simulink model "RealseCheckPWMController"  (R2026a)
settings: Solver=ode4  StopTime=inf  FixedStep=1/500  EnableMultiTasking=on
undefined symbols (not defined in the file): HIL, qc_get_step_size
libraries: quarc_library x12
settings Model: SimulationMode=external  ExtModeTrigDuration=10000  Creator=fvranes  LastModifiedBy=meow1
settings SolverCC: PositivePriorityOrder=on
settings RTWCC: SystemTargetFile=quarc_win64.tlc  TemplateMakefile=quarc_default_tmf  Toolchain=QUARC win64 | nmake (64-bit Windows)  BuildConfiguration=Faster Runs  Description=QUARC Win64 Target Using Toolchain
settings STFCustomTargetCC: SystemTargetFile=quarc_win64.tlc  MultiwordLength=2048.0  ConcurrentExecutionCompliant=on  UseToolchainInfoCompliant=on
settings GRTTargetCC: ExtMode=on  ExtModeMexFile=quarc_comm  ParMdlRefBuildCompliant=off  CompOptLevelCompliant=off  CombineOutputUpdateFcns=off  MatFileLogging=off  CPPClassGenCompliant=off  GRTInterface=on
settings ConfigComp: CovMetricSettings=dswe

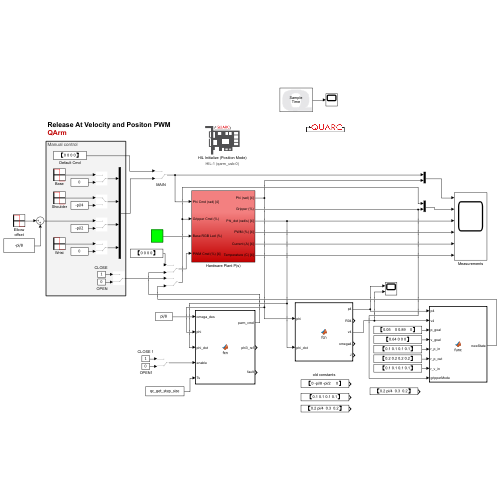
[thumbnail: Simulink's stored preview of the top-level diagram]
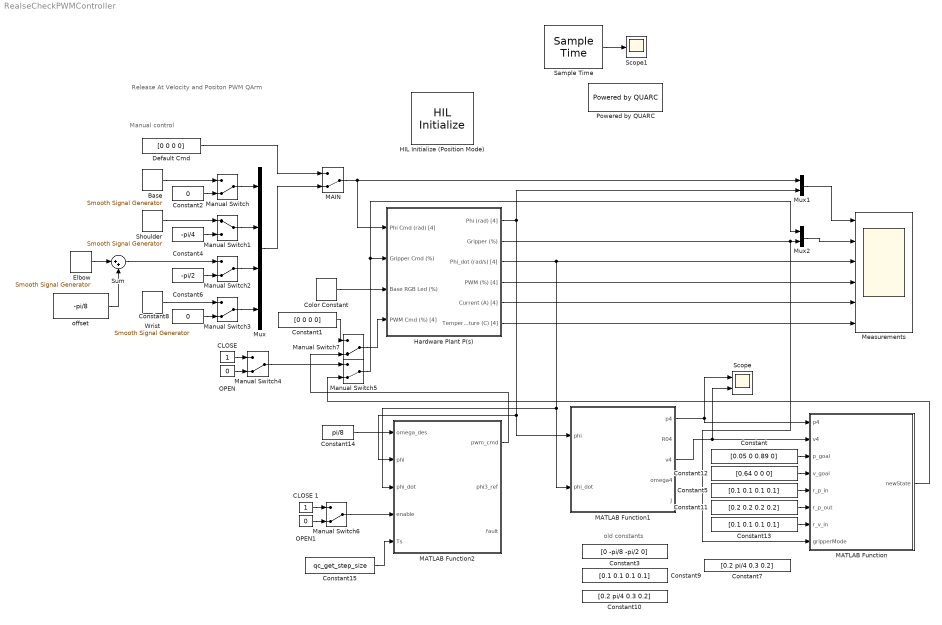
== system RealseCheckPWMController ==
  note: old constants
  note: Manual control
  note: Release At Velocity and Positon PWM
      | QArm
  " OPEN" : Constant  Value=0
  " OPEN1" : Constant  Value=0
  Base : quarc_library/Sources/Signals/Smooth Signal Generator  signal_type=Square  source=Internal (dialog parameters)  amplitude=pi/8  frequency=0.125  initial_phase=0  sample_time=qc_get_step_size  output_cos=off
      settings: SourceProductName=QUARC Targets
  "CLOSE " : Constant
  CLOSE 1 : Constant
  Color Constant : quarc_library/Sources/Signals/Color Constant  color=[0 1 0]
      settings: SourceProductName=QUARC Targets
  Constant : Constant  Value=[0.05 0 0.89 0]
  Constant1 : Constant  Value=[0 0 0 0]
  Constant10 : Constant  Value=[0.2 pi/4 0.3 0.2]
  Constant11 : Constant  Value=[0.2 0.2 0.2 0.2]
  Constant12 : Constant  Value=[0.64 0 0 0]
  Constant13 : Constant  Value=[0.1 0.1 0.1 0.1]
  Constant14 : Constant  Value=pi/8
  Constant15 : Constant  Value=qc_get_step_size
  Constant2 : Constant  Value=0
  Constant3 : Constant  Value=[0 -pi/8 -pi/2 0]
  Constant4 : Constant  Value=-pi/4
  Constant5 : Constant  Value=[0.1 0.1 0.1 0.1]
  Constant6 : Constant  Value=-pi/2
  Constant7 : Constant  Value=[0.2 pi/4 0.3 0.2]
  Constant8 : Constant  Value=0
  Constant9 : Constant  Value=[0.1 0.1 0.1 0.1]
  Default Cmd : Constant  Value=[0 0 0 0]
  Elbow : quarc_library/Sources/Signals/Smooth Signal Generator  signal_type=Square  source=Internal (dialog parameters)  amplitude=pi/4  frequency=0.25  initial_phase=pi  sample_time=qc_get_step_size  output_cos=off
      settings: SourceProductName=QUARC Targets
  HIL Initialize (Position Mode) : quarc_library/Data Acquisition/Generic/Configuration/HIL Initialize  object_name=HIL-1  board_type=qarm_usb  board_number=0  board_options=j0_mode=0;j1_mode=0;j2_mode=1;j3_mode=0;gripper_mode=0;j0_profile_config=0;j0_profile_velocity=1.6;j0_profile_acceleration=1.0472;j1_profile_config=0;j1_profile_velocity=1.6;j1_profile_acceleration=1.0472;j2_profile_config=0;j2_profile_velocity=1.6;j2_profile_acceleration=1.0472;j3_profile_config=0;j3_profile_velocity=1.6;j3_profile_acceleration=1.0472;  exclusive=off  active=on  hardware_clocks=[0]  clock_modes=[]  initial_clock_frequencies=[]  set_clock_params_at_start=off  set_clock_params_at_switch_in=off  set_clock_frequencies_at_start=off  set_clock_frequencies_at_switch_in=off  analog_input_channels=[5:9]  analog_input_configurations=[]  analog_input_maximums=[]  analog_input_minimums=[]  set_analog_input_params_at_start=off  set_analog_input_params_at_switch_in=off  analog_output_channels=[]  analog_output_maximums=inf  analog_output_minimums=-inf  initial_analog_outputs=[0]  final_analog_outputs=[0]  watchdog_analog_outputs=[]  set_analog_output_params_at_start=off  set_analog_output_params_at_switch_in=off  set_analog_outputs_at_start=off  set_analog_outputs_at_switch_in=off  set_analog_outputs_at_terminate=off  set_analog_outputs_at_switch_out=off  set_analog_outputs_on_watchdog=off  digital_input_channels=[]  digital_output_channels=[]  digital_output_configuration=[]  initial_digital_outputs=[0]  final_digital_outputs=[0]  watchdog_digital_outputs=[0]  set_digital_output_params_at_start=off  set_digital_output_params_at_switch_in=off  set_digital_outputs_at_start=off  set_digital_outputs_at_switch_in=off  set_digital_outputs_at_terminate=off  set_digital_outputs_at_switch_out=off  set_digital_outputs_on_watchdog=off  encoder_channels=[]  quadrature=[]  encoder_filter_frequency=[]  initial_encoder_counts=[]  set_encoder_params_at_start=off  set_encoder_params_at_switch_in=off  set_encoder_counts_at_start=off  set_encoder_counts_at_switch_in=off  pwm_channels=[]  pwm_modes=[]  pwm_frequency=[]  pwm_configuration=[]  pwm_alignment=[]  pwm_polarity=[]  pwm_leading_deadband=[]  pwm_trailing_deadband=[]  initial_pwm_outputs=[]  final_pwm_outputs=[]  watchdog_pwm_outputs=[]  set_pwm_params_at_start=off  set_pwm_params_at_switch_in=off  set_pwm_outputs_at_start=off  set_pwm_outputs_at_switch_in=off  set_pwm_outputs_at_terminate=off  set_pwm_outputs_at_switch_out=off  set_pwm_outputs_on_watchdog=off  other_output_channels=[11005:11008 1000:1004 11000:11003]  initial_other_outputs=[zeros(1,9), ones(1,3)]  final_other_outputs=[1 0 0 0]  watchdog_other_outputs=zeros(1,12)  set_other_outputs_at_start=off  set_other_outputs_at_switch_in=off  set_other_outputs_at_terminate=on  set_other_outputs_at_switch_out=off  set_other_outputs_on_watchdog=off
  Hardware Plant P(s) : Subsystem
  MAIN : ManualSwitch  CurrentSetting=0
  MATLAB Function : MATLAB Function  TreatAsAtomicUnit=on
  MATLAB Function1 : MATLAB Function  TreatAsAtomicUnit=on
  MATLAB Function2 : MATLAB Function  TreatAsAtomicUnit=on
  Manual Switch{,2..7} (7 alike) : ManualSwitch  CurrentSetting=0
  Manual Switch1 : ManualSwitch
  Measurements : Scope  NumInputPorts=6
      settings: TimeSpan=20  Title=Phi (angular position)  ActiveDisplayYMinimum=-3.0435003762492152  ActiveDisplayYMaximum=0.767085796973318  YLabel=degrees
  Mux : Mux
  Mux1 : Mux  Inputs=2
  Mux2 : Mux  Inputs=2
  Powered by QUARC : quarc_library/Logos/Powered by QUARC
  Sample Time : quarc_library/Sources/Time/Sample Time  Priority=-99  sample_time=qc_get_step_size
  Scope : Scope  NumInputPorts=2
      settings: DataLoggingVariableName=ScopeData2
  Scope1 : Scope
      settings: ActiveDisplayYMinimum=0.00125  ActiveDisplayYMaximum=0.00274
  Shoulder : quarc_library/Sources/Signals/Smooth Signal Generator  signal_type=Square  source=Internal (dialog parameters)  amplitude=pi/3  frequency=0.25  initial_phase=0  sample_time=qc_get_step_size  output_cos=off
      settings: SourceProductName=QUARC Targets
  Sum : Sum  Inputs=|++
  Wrist : quarc_library/Sources/Signals/Smooth Signal Generator  signal_type=Square  source=Internal (dialog parameters)  amplitude=pi/8  frequency=0.125  initial_phase=0  sample_time=qc_get_step_size  output_cos=off
      settings: SourceProductName=QUARC Targets
  offset : Constant  Value=-pi/8
  wires:
  Color Constant/1 -> Hardware Plant P(s)/3(Base RGB Led (%))
  Constant2/1 -> Manual Switch/2
  Constant4/1 -> Manual Switch1/2
  Constant6/1 -> Manual Switch2/2
  Constant8/1 -> Manual Switch3/2
  Wrist/1 -> Manual Switch3/1
  Manual Switch2/1 -> Mux/3
  Manual Switch3/1 -> Mux/4
  Manual Switch1/1 -> Mux/2
  Manual Switch/1 -> Mux/1
  Mux/1 -> MAIN/2
  Default Cmd/1 -> MAIN/1
  MAIN/1 -> Mux1/1, Hardware Plant P(s)/1(Phi Cmd (rad) [4])
  "CLOSE "/1 -> Manual Switch4/1
  Base/1 -> Manual Switch/1
  Shoulder/1 -> Manual Switch1/1
  Elbow/1 -> Sum/1
  Sample Time/1 -> Scope1/1
  " OPEN"/1 -> Manual Switch4/2
  Hardware Plant P(s)/2(Gripper (%)) -> Mux2/2, MATLAB Function/8(gripperMode)
  Constant/1 -> MATLAB Function/3(p_goal)
  Constant5/1 -> MATLAB Function/5(r_p_in)
  Hardware Plant P(s)/1(Phi (rad) [4]) -> MATLAB Function2/2(phi), MATLAB Function1/1(phi), Mux1/2
  Hardware Plant P(s)/3(Phi_dot (rad/s) [4]) -> MATLAB Function1/2(phi_dot), MATLAB Function2/3(phi_dot), Measurements/3
  Mux2/1 -> Measurements/2
  Mux1/1 -> Measurements/1
  Hardware Plant P(s)/4(PWM (%) [4]) -> Measurements/4
  Hardware Plant P(s)/5(Current (A) [4]) -> Measurements/5
  Hardware Plant P(s)/6(Temperature (C) [4]) -> Measurements/6
  Manual Switch4/1 -> Manual Switch5/1
  MATLAB Function/1(newState) -> Manual Switch5/2
  Manual Switch5/1 -> Mux2/1, Hardware Plant P(s)/2(Gripper Cmd (%))
  offset/1 -> Sum/2
  Sum/1 -> Manual Switch2/1
  MATLAB Function1/1(p4) -> Scope/1, MATLAB Function/1(p4)
  MATLAB Function1/3(v4) -> Scope/2, MATLAB Function/2(v4)
  Constant11/1 -> MATLAB Function/6(r_p_out)
  Constant12/1 -> MATLAB Function/4(v_goal)
  Constant13/1 -> MATLAB Function/7(r_v_in)
  Constant14/1 -> MATLAB Function2/1(omega_des)
  CLOSE 1/1 -> Manual Switch6/1
  " OPEN1"/1 -> Manual Switch6/2
  Manual Switch6/1 -> MATLAB Function2/4(enable)
  Constant1/1 -> Manual Switch7/1
  MATLAB Function2/1(pwm_cmd) -> Manual Switch7/2
  Manual Switch7/1 -> Hardware Plant P(s)/4(PWM Cmd (%) [4])
  Constant15/1 -> MATLAB Function2/5(Ts)

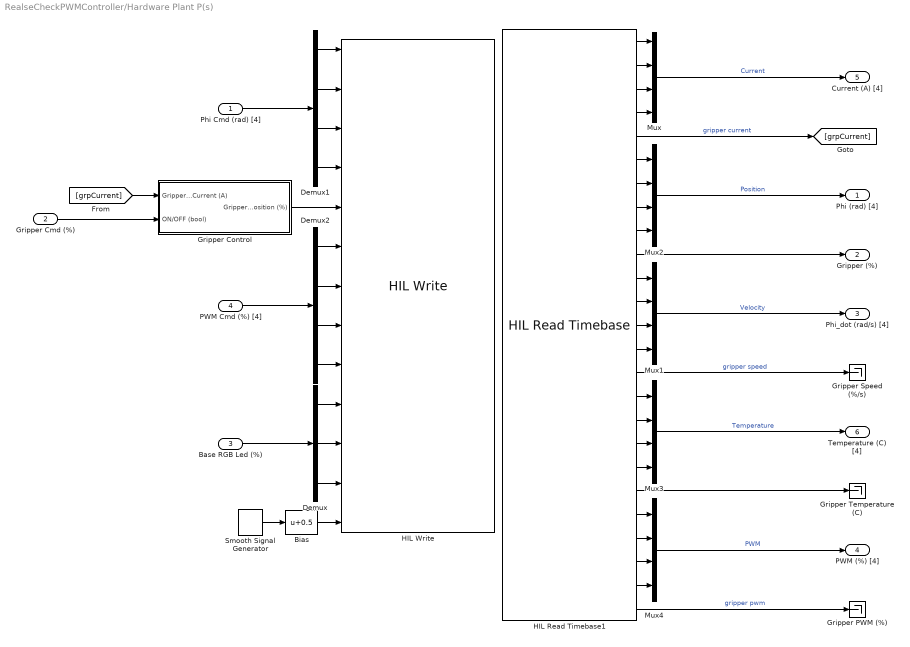
== system RealseCheckPWMController/Hardware Plant P(s) ==
  Phi Cmd (rad) [4] : Inport
  Gripper Cmd (%) : Inport  Port=2
  Base RGB Led (%) : Inport  Port=3
  PWM Cmd (%) [4] : Inport  Port=4
  Bias : Bias  Bias=0.5  SaturateOnIntegerOverflow=off
  Demux : Demux  Outputs=3
  Demux1 : Demux
  Demux2 : Demux
  Gripper Control : Subsystem
  Gripper PWM (%) : Terminator
  Gripper Speed (%/s) : Terminator
  Gripper Temperature (C) : Terminator
  HIL Read Timebase1 : quarc_library/Data Acquisition/Generic/Timebases/HIL Read Timebase  object_name=HIL-1  clock=0  analog_channels=[5:9]  encoder_channels=[]  digital_channels=[]  other_channels=[1000:1004 3000:3004 10000:10004 11000:11004]  active=on  vector_output=off  port_labels=channel numbers  data_type_mode=Inherit via back propagation  encoder_data_type=double  digital_data_type=boolean  overflow_mode=Error on overflow  samples_in_buffer=max(ceil(1/qc_get_step_size), 1)
  HIL Write : quarc_library/Data Acquisition/Generic/Immediate I//O/HIL Write  object_name=HIL-1  analog_channels=[]  pwm_channels=[]  digital_channels=[]  other_channels=[1000:1004 11000:11003 11005:11008]  sample_time=-1  active=on  vector_input=off  port_labels=channel numbers
  Mux{,1..4} (5 alike) : Mux
  Smooth Signal Generator : quarc_library/Sources/Signals/Smooth Signal Generator  signal_type=Sine  source=Internal (dialog parameters)  amplitude=0.5  frequency=0.5  initial_phase=0  sample_time=qc_get_step_size  output_cos=off
      settings: SourceProductName=QUARC Targets
  Phi (rad) [4] : Outport  VectorParamsAs1DForOutWhenUnconnected=off
  Gripper (%) : Outport  Port=2  VectorParamsAs1DForOutWhenUnconnected=off
  Phi_dot (rad/s) [4] : Outport  Port=3  VectorParamsAs1DForOutWhenUnconnected=off
  PWM (%) [4] : Outport  Port=4  VectorParamsAs1DForOutWhenUnconnected=off
  Current (A) [4] : Outport  Port=5  VectorParamsAs1DForOutWhenUnconnected=off
  Temperature (C) [4] : Outport  Port=6  VectorParamsAs1DForOutWhenUnconnected=off
  wires:
  Gripper Cmd (%)/1 -> Gripper Control/2(ON/OFF (bool))
  HIL Read Timebase1/10 -> Gripper (%)/1
  Mux4/1 -> PWM (%) [4]/1  "PWM"
  HIL Read Timebase1/25 -> Gripper PWM (%)/1  "gripper pwm"
  HIL Read Timebase1/24 -> Mux4/4
  HIL Read Timebase1/23 -> Mux4/3
  HIL Read Timebase1/22 -> Mux4/2
  HIL Read Timebase1/21 -> Mux4/1
  Mux2/1 -> Phi (rad) [4]/1  "Position"
  Demux2/4 -> HIL Write/9
  Demux2/3 -> HIL Write/8
  Demux2/2 -> HIL Write/7
  Demux2/1 -> HIL Write/6
  PWM Cmd (%) [4]/1 -> Demux2/1
  Phi Cmd (rad) [4]/1 -> Demux1/1
  Demux1/4 -> HIL Write/4
  Demux1/3 -> HIL Write/3
  Demux1/2 -> HIL Write/2
  Demux1/1 -> HIL Write/1
  Base RGB Led (%)/1 -> Demux/1
  Mux3/1 -> Temperature (C) [4]/1  "Temperature"
  Mux1/1 -> Phi_dot (rad/s) [4]/1  "Velocity"
  Mux/1 -> Current (A) [4]/1  "Current"
  HIL Read Timebase1/20 -> Gripper Temperature (C)/1
  HIL Read Timebase1/1 -> Mux/1
  HIL Read Timebase1/2 -> Mux/2
  HIL Read Timebase1/13 -> Mux1/3
  Demux/2 -> HIL Write/11
  HIL Read Timebase1/19 -> Mux3/4
  Demux/1 -> HIL Write/10
  HIL Read Timebase1/11 -> Mux1/1
  HIL Read Timebase1/16 -> Mux3/1
  HIL Read Timebase1/17 -> Mux3/2
  HIL Read Timebase1/3 -> Mux/3
  Demux/3 -> HIL Write/12
  HIL Read Timebase1/15 -> Gripper Speed (%/s)/1  "gripper speed"
  HIL Read Timebase1/5 -> [grpCurrent]  "gripper current"
  HIL Read Timebase1/7 -> Mux2/2
  HIL Read Timebase1/4 -> Mux/4
  HIL Read Timebase1/12 -> Mux1/2
  HIL Read Timebase1/8 -> Mux2/3
  HIL Read Timebase1/18 -> Mux3/3
  HIL Read Timebase1/6 -> Mux2/1
  HIL Read Timebase1/9 -> Mux2/4
  HIL Read Timebase1/14 -> Mux1/4
  Smooth Signal Generator/1 -> Bias/1
  Bias/1 -> HIL Write/13
  Gripper Control/1(Gripper Position (%)) -> HIL Write/5
  [grpCurrent] -> Gripper Control/1(Gripper Current (A))

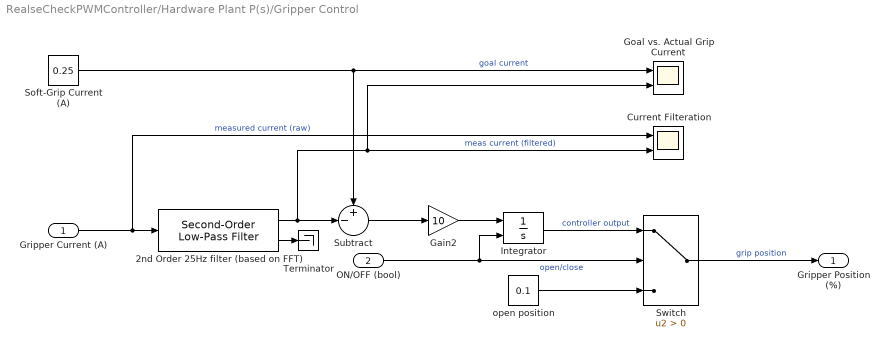
== system RealseCheckPWMController/Hardware Plant P(s)/Gripper Control ==
  Gripper Current (A) : Inport
  ON/OFF (bool) : Inport  Port=2
  2nd Order 25Hz filter (based on FFT) : quarc_library/Continuous/Second-Order Low-Pass Filter  params_source=Internal (dialog parameters)  input_width=25*2*pi  input_zeta=1  input_init=0
  Current Filteration : Scope  NumInputPorts=2
      settings: ActiveDisplayYMinimum=-0.01447  ActiveDisplayYMaximum=0.62651  DataLoggingVariableName=ScopeData5
  Gain2 : Gain  Gain=10
  Goal vs. Actual Grip Current : Scope  NumInputPorts=2
      settings: ActiveDisplayYMinimum=0.00229  ActiveDisplayYMaximum=0.27702  DataLoggingVariableName=ScopeData4
  Integrator : Integrator  ExternalReset=either  InitialCondition=0.1  LimitOutput=on  UpperSaturationLimit=0.9  LowerSaturationLimit=0.1
  Soft-Grip Current (A) : Constant  Value=0.25
  Subtract : Sum  Inputs=+-|
  Switch : Switch  Criteria=u2 > Threshold  SaturateOnIntegerOverflow=off  InputSameDT=off
  Terminator : Terminator
  open position : Constant  Value=0.1
  Gripper Position (%) : Outport  VectorParamsAs1DForOutWhenUnconnected=off
  wires:
  Gripper Current (A)/1 -> 2nd Order 25Hz filter (based on FFT)/1, Current Filteration/1  "measured current (raw)"
  ON/OFF (bool)/1 -> Switch/2, Integrator/2  "open/close"
  open position/1 -> Switch/3
  Switch/1 -> Gripper Position (%)/1  "grip position"
  Soft-Grip Current (A)/1 -> Subtract/1, Goal vs. Actual Grip Current/1  "goal current"
  2nd Order 25Hz filter (based on FFT)/1 -> Subtract/2, Current Filteration/2, Goal vs. Actual Grip Current/2  "meas current (filtered)"
  Subtract/1 -> Gain2/1
  Integrator/1 -> Switch/1  "controller output"
  Gain2/1 -> Integrator/1
  2nd Order 25Hz filter (based on FFT)/2 -> Terminator/1

== matlab function RealseCheckPWMController/MATLAB Function1 ==
  data: phi input; p4 output; R04 output; v4 output; omega4 output; J output; phi_dot input
function [p4, R04, v4, omega4, J] = fcn(phi, phi_dot)
[p4, R04, v4, omega4, J] = qarmForwardKinematics(phi, phi_dot)

== matlab function RealseCheckPWMController/MATLAB Function ==
  data: p4 input; v4 input; newState output; p_goal input; v_goal input; r_p_in input; r_p_out input; r_v_in input; gripperMode input
function newState = func(p4, v4, p_goal, v_goal, r_p_in, r_p_out, r_v_in, gripperMode)
newState = ReleaseCheck(p4, v4, p_goal, v_goal, r_p_in, r_p_out, r_v_in, gripperMode)

== matlab function RealseCheckPWMController/MATLAB Function2 ==
  data: omega_des input; pwm_cmd output; phi input; phi_dot input; enable input; Ts input; phi3_ref output; fault output
function [pwm_cmd, phi3_ref, fault] = fcn(omega_des, phi, phi_dot, enable, Ts)
[pwm_cmd, phi3_ref, fault] = ElbowSpeedControl(omega_des, phi, phi_dot, enable, Ts);
